simulink model "dual_thyristor_bridge_rectifier"  (R2025b)
settings: Solver=ode1be  StartTime=0.0  StopTime=simlength  FixedStep=tc  MaxStep=tc
values from neighbouring files (symbols this model uses):
  n1 = 35    [voltage_spectrum_analysis.m]
  omega_grid_emulator_nom = w_grid    (= 314.159265359)    [grid_emulator.m]
  vn_eta_pu = 0    [grid_emulator.m]
  vn_xi_pu = 0    [grid_emulator.m]
  vp_xi_pu = 1    [grid_emulator.m]
  w_grid = f_grid*2*pi    (= 314.159265359)    [grid_emulator.m]
undefined symbols (not defined in the file or in its folder): CSF_11, CSF_13, CSF_5, CSF_7, delta_fht1, Idc_traction_normalization_factor, ki_u_ctrl, kp_u_ctrl, Ld_fht1, LFu_dc, LSF_11, LSF_13, LSF_5, LSF_7, magnitude, n10, omega_fht1, pll_i1, pll_p, RLFu_dc, tc, Tcontrol_rect, ts_ctrl_rect, ugrid_factor, Vdc_traction_normalization_factor, Vgrid_phase_normalization_factor
libraries: fl_lib x299, nesl_utility x67, ee_lib x24, single_phase_transformer_lib x3, cstblocks x3
(part 6 of 6)

== system dual_thyristor_bridge_rectifier/dual_rectifier_bridge/neg_bridge/firing3/oscillator ==
  Data Type Conversion : DataTypeConversion  OutDataTypeStr=double  SaturateOnIntegerOverflow=off  RndMeth=Floor
  Logical Operator1 : Logic  Operator=NOT  AllPortsSameDT=off  OutDataTypeStr=boolean
  Rate Transition : RateTransition  OutPortSampleTime=ts
  Simulink-PS Converter : nesl_utility/Simulink-PS Converter  PhysicalDomain=network_engine_domain  SubClassName=ps_input  LeftPortType=input  RightPortType=output  PseudoPeriodic=off  Frequencies=[]  NoiseDistribution=none  NoiseParameters=[]  Unit=1  AffineConversion=off  FilteringAndDerivatives=provide  SimscapeFilterOrder=1  InputFilterTimeConstant=0.001  UdotUserProvided=0
  Unit Delay1 : UnitDelay  SampleTime=Tcontrol_rect  HasFrameUpgradeWarning=on
  output : PMIOPort  Side=Right
  wires:
  Data Type Conversion/1 -> Rate Transition/1
  Unit Delay1/1 -> Logical Operator1/1
  Logical Operator1/1 -> Unit Delay1/1, Data Type Conversion/1
  Rate Transition/1 -> Simulink-PS Converter/1
  connections:
  Simulink-PS Converter/RConn1 -- output/RConn1

== system dual_thyristor_bridge_rectifier/dual_rectifier_bridge/neg_bridge/firing4/oscillator ==
  Data Type Conversion : DataTypeConversion  OutDataTypeStr=double  SaturateOnIntegerOverflow=off  RndMeth=Floor
  Logical Operator1 : Logic  Operator=NOT  AllPortsSameDT=off  OutDataTypeStr=boolean
  Rate Transition : RateTransition  OutPortSampleTime=ts
  Simulink-PS Converter : nesl_utility/Simulink-PS Converter  PhysicalDomain=network_engine_domain  SubClassName=ps_input  LeftPortType=input  RightPortType=output  PseudoPeriodic=off  Frequencies=[]  NoiseDistribution=none  NoiseParameters=[]  Unit=1  AffineConversion=off  FilteringAndDerivatives=provide  SimscapeFilterOrder=1  InputFilterTimeConstant=0.001  UdotUserProvided=0
  Unit Delay1 : UnitDelay  SampleTime=Tcontrol_rect  HasFrameUpgradeWarning=on
  output : PMIOPort  Side=Right
  wires:
  Logical Operator1/1 -> Unit Delay1/1, Data Type Conversion/1
  Unit Delay1/1 -> Logical Operator1/1
  Data Type Conversion/1 -> Rate Transition/1
  Rate Transition/1 -> Simulink-PS Converter/1
  connections:
  Simulink-PS Converter/RConn1 -- output/RConn1

== system dual_thyristor_bridge_rectifier/dual_rectifier_bridge/neg_bridge/firing5/oscillator ==
  Data Type Conversion : DataTypeConversion  OutDataTypeStr=double  SaturateOnIntegerOverflow=off  RndMeth=Floor
  Logical Operator1 : Logic  Operator=NOT  AllPortsSameDT=off  OutDataTypeStr=boolean
  Rate Transition : RateTransition  OutPortSampleTime=ts
  Simulink-PS Converter : nesl_utility/Simulink-PS Converter  PhysicalDomain=network_engine_domain  SubClassName=ps_input  LeftPortType=input  RightPortType=output  PseudoPeriodic=off  Frequencies=[]  NoiseDistribution=none  NoiseParameters=[]  Unit=1  AffineConversion=off  FilteringAndDerivatives=provide  SimscapeFilterOrder=1  InputFilterTimeConstant=0.001  UdotUserProvided=0
  Unit Delay1 : UnitDelay  SampleTime=Tcontrol_rect  HasFrameUpgradeWarning=on
  output : PMIOPort  Side=Right
  wires:
  Data Type Conversion/1 -> Rate Transition/1
  Unit Delay1/1 -> Logical Operator1/1
  Logical Operator1/1 -> Unit Delay1/1, Data Type Conversion/1
  Rate Transition/1 -> Simulink-PS Converter/1
  connections:
  Simulink-PS Converter/RConn1 -- output/RConn1

== system dual_thyristor_bridge_rectifier/dual_rectifier_bridge/neg_bridge/firing6/oscillator ==
  Data Type Conversion : DataTypeConversion  OutDataTypeStr=double  SaturateOnIntegerOverflow=off  RndMeth=Floor
  Logical Operator1 : Logic  Operator=NOT  AllPortsSameDT=off  OutDataTypeStr=boolean
  Rate Transition : RateTransition  OutPortSampleTime=ts
  Simulink-PS Converter : nesl_utility/Simulink-PS Converter  PhysicalDomain=network_engine_domain  SubClassName=ps_input  LeftPortType=input  RightPortType=output  PseudoPeriodic=off  Frequencies=[]  NoiseDistribution=none  NoiseParameters=[]  Unit=1  AffineConversion=off  FilteringAndDerivatives=provide  SimscapeFilterOrder=1  InputFilterTimeConstant=0.001  UdotUserProvided=0
  Unit Delay1 : UnitDelay  SampleTime=Tcontrol_rect  HasFrameUpgradeWarning=on
  output : PMIOPort  Side=Right
  wires:
  Logical Operator1/1 -> Data Type Conversion/1, Unit Delay1/1
  Unit Delay1/1 -> Logical Operator1/1
  Data Type Conversion/1 -> Rate Transition/1
  Rate Transition/1 -> Simulink-PS Converter/1
  connections:
  Simulink-PS Converter/RConn1 -- output/RConn1

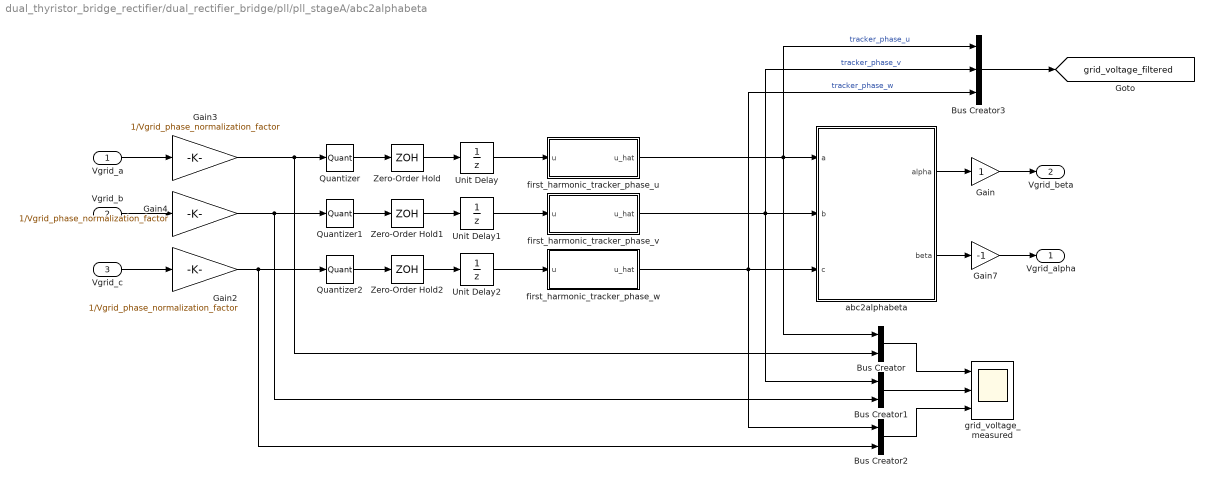
== system dual_thyristor_bridge_rectifier/dual_rectifier_bridge/pll/pll_stageA/abc2alphabeta ==
  Vgrid_a : Inport
  Vgrid_b : Inport  Port=2
  Vgrid_c : Inport  Port=3
  Bus Creator : BusCreator  Inputs=2
  Bus Creator1 : BusCreator  Inputs=2
  Bus Creator2 : BusCreator  Inputs=2
  Bus Creator3 : BusCreator  Inputs=3
  Gain : Gain
  Gain2 : Gain  Gain=1/Vgrid_phase_normalization_factor
  Gain3 : Gain  Gain=1/Vgrid_phase_normalization_factor
  Gain4 : Gain  Gain=1/Vgrid_phase_normalization_factor
  Gain7 : Gain  Gain=-1
  Quantizer : Quantizer  QuantizationInterval=2^-11
  Quantizer1 : Quantizer  QuantizationInterval=2^-11
  Quantizer2 : Quantizer  QuantizationInterval=2^-11
  Unit Delay : UnitDelay  SampleTime=ts_ctrl_rect  HasFrameUpgradeWarning=on
  Unit Delay1 : UnitDelay  SampleTime=ts_ctrl_rect  HasFrameUpgradeWarning=on
  Unit Delay2 : UnitDelay  SampleTime=ts_ctrl_rect  HasFrameUpgradeWarning=on
  Zero-Order Hold : ZeroOrderHold  SampleTime=ts_ctrl_rect
  Zero-Order Hold1 : ZeroOrderHold  SampleTime=ts_ctrl_rect
  Zero-Order Hold2 : ZeroOrderHold  SampleTime=ts_ctrl_rect
  abc2alphabeta : Subsystem
  first_harmonic_tracker_phase_u : Subsystem
  first_harmonic_tracker_phase_v : Subsystem
  first_harmonic_tracker_phase_w : Subsystem
  grid_voltage_measured : Scope  NumInputPorts=3
      settings: SampleTime=ts_ctrl_rect  ActiveDisplayYMinimum=-1.64432  ActiveDisplayYMaximum=1.33618
  Vgrid_alpha : Outport
  Vgrid_beta : Outport  Port=2
  tag scope: grid_voltage_filtered=global
  wires:
  Vgrid_a/1 -> Gain3/1
  Vgrid_b/1 -> Gain4/1
  Vgrid_c/1 -> Gain2/1
  abc2alphabeta/2("beta ") -> Gain7/1
  abc2alphabeta/1("alpha ") -> Gain/1
  Gain/1 -> Vgrid_beta/1
  Gain7/1 -> Vgrid_alpha/1
  Zero-Order Hold/1 -> Unit Delay/1
  Zero-Order Hold1/1 -> Unit Delay1/1
  Zero-Order Hold2/1 -> Unit Delay2/1
  Bus Creator3/1 -> [grid_voltage_filtered]
  Bus Creator/1 -> grid_voltage_measured/1
  Bus Creator1/1 -> grid_voltage_measured/2
  Bus Creator2/1 -> grid_voltage_measured/3
  first_harmonic_tracker_phase_u/1(u_hat) -> Bus Creator/1, Bus Creator3/1, abc2alphabeta/1(a)  "tracker_phase_u"
  first_harmonic_tracker_phase_v/1(u_hat) -> Bus Creator1/1, Bus Creator3/2, abc2alphabeta/2(b)  "tracker_phase_v"
  first_harmonic_tracker_phase_w/1(u_hat) -> Bus Creator2/1, abc2alphabeta/3(c), Bus Creator3/3  "tracker_phase_w"
  Unit Delay1/1 -> first_harmonic_tracker_phase_v/1(u)
  Unit Delay/1 -> first_harmonic_tracker_phase_u/1(u)
  Unit Delay2/1 -> first_harmonic_tracker_phase_w/1(u)
  Gain3/1 -> Quantizer/1, Bus Creator/2
  Gain4/1 -> Quantizer1/1, Bus Creator1/2
  Gain2/1 -> Quantizer2/1, Bus Creator2/2
  Quantizer2/1 -> Zero-Order Hold2/1
  Quantizer1/1 -> Zero-Order Hold1/1
  Quantizer/1 -> Zero-Order Hold/1

== system dual_thyristor_bridge_rectifier/dual_rectifier_bridge/pll/pll_stageB/alphabeta2xieta ==
  alpha : Inport
  beta : Inport  Port=2
  wt : Inport  Port=3
  Product{,1..3} (4 alike) : Product  RndMeth=Zero
  Sum : Sum
  Sum1 : Sum  Inputs=-+
  Trigonometric Function : Trigonometry  Operator=cos
  Trigonometric Function1 : Trigonometry
  xi : Outport
  eta : Outport  Port=2
  wires:
  Trigonometric Function/1 -> [cos]
  Trigonometric Function1/1 -> [sin]
  wt/1 -> Trigonometric Function1/1, Trigonometric Function/1
  Sum1/1 -> eta/1
  Sum/1 -> xi/1
  [cos] -> Product3/1
  Product3/1 -> Sum1/2
  Product2/1 -> Sum1/1
  [sin] -> Product2/1
  beta/1 -> Product3/2, Product1/2
  [sin] -> Product1/1
  Product1/1 -> Sum/2
  Product/1 -> Sum/1
  alpha/1 -> Product2/2, Product/2
  [cos] -> Product/1

== system dual_thyristor_bridge_rectifier/dual_rectifier_bridge/pll/pll_stageB/pll_2 ==
  eta : Inport
  -2<x<2 : Saturate  UpperLimit=2  LowerLimit=-2
  Constant1 : Constant  Value=2*pi
  Constant3 : Constant  Value=0
  Constant4 : Constant  Value=w_grid
  Constant7 : Constant
  Math Function1 : Math  Operator=mod  SignedPower=on
  Product1 : Product  RndMeth=Zero
  Product2 : Product  RndMeth=Zero
  Sum1 : Sum  Inputs=|-+
  Sum3 : Sum  SaturateOnIntegerOverflow=on
  Sum4 : Sum  SaturateOnIntegerOverflow=on
  Sum5 : Sum  Inputs=+++
  Unit Delay1 : UnitDelay  SampleTime=ts_ctrl_rect  HasFrameUpgradeWarning=on
  Unit Delay4 : UnitDelay  SampleTime=ts_ctrl_rect  HasFrameUpgradeWarning=on
  kp : Gain  Gain=pll_i1*ts_ctrl_rect  SaturateOnIntegerOverflow=on  OutDataTypeStr=Inherit: Same as input  ParamDataTypeStr=Inherit: Same as input
  kp1 : Gain  Gain=pll_p  SaturateOnIntegerOverflow=on  OutDataTypeStr=Inherit: Same as input  ParamDataTypeStr=Inherit: Same as input
  kp2 : Gain  Gain=ts_ctrl_rect  SaturateOnIntegerOverflow=on  OutDataTypeStr=Inherit: Same as input  ParamDataTypeStr=Inherit: Same as input
  kp3 : Gain  Gain=-1  SaturateOnIntegerOverflow=on  OutDataTypeStr=Inherit: Same as input  ParamDataTypeStr=Inherit: Same as input
  theta_est : Outport
  wires:
  Constant7/1 -> Sum5/3
  Constant3/1 -> Sum1/2
  [Vgrid_unorm_posneg] -> Product1/2
  Product2/1 -> kp2/1
  kp/1 -> Sum3/1
  Sum4/1 -> Math Function1/1
  kp1/1 -> Sum5/1
  Product1/1 -> Sum1/1
  Sum1/1 -> kp3/1
  Math Function1/1 -> theta_est/1, Unit Delay1/1
  -2<x<2/1 -> Unit Delay4/1, Sum5/2  "i1"
  Unit Delay4/1 -> Sum3/2
  Sum3/1 -> -2<x<2/1
  kp2/1 -> Sum4/1
  Sum5/1 -> Product2/1
  Constant4/1 -> Product2/2
  Unit Delay1/1 -> Sum4/2
  Constant1/1 -> Math Function1/2
  eta/1 -> Product1/1
  kp3/1 -> kp/1, kp1/1

== system dual_thyristor_bridge_rectifier/dual_rectifier_bridge/pos_bridge/firing1/oscillator ==
  Data Type Conversion : DataTypeConversion  OutDataTypeStr=double  SaturateOnIntegerOverflow=off  RndMeth=Floor
  Logical Operator1 : Logic  Operator=NOT  AllPortsSameDT=off  OutDataTypeStr=boolean
  Rate Transition : RateTransition  OutPortSampleTime=ts
  Simulink-PS Converter : nesl_utility/Simulink-PS Converter  PhysicalDomain=network_engine_domain  SubClassName=ps_input  LeftPortType=input  RightPortType=output  PseudoPeriodic=off  Frequencies=[]  NoiseDistribution=none  NoiseParameters=[]  Unit=1  AffineConversion=off  FilteringAndDerivatives=provide  SimscapeFilterOrder=1  InputFilterTimeConstant=0.001  UdotUserProvided=0
  Unit Delay1 : UnitDelay  SampleTime=Tcontrol_rect  HasFrameUpgradeWarning=on
  output : PMIOPort  Side=Right
  wires:
  Rate Transition/1 -> Simulink-PS Converter/1
  Logical Operator1/1 -> Data Type Conversion/1, Unit Delay1/1
  Unit Delay1/1 -> Logical Operator1/1
  Data Type Conversion/1 -> Rate Transition/1
  connections:
  Simulink-PS Converter/RConn1 -- output/RConn1

== system dual_thyristor_bridge_rectifier/dual_rectifier_bridge/pos_bridge/firing2/oscillator ==
  Data Type Conversion : DataTypeConversion  OutDataTypeStr=double  SaturateOnIntegerOverflow=off  RndMeth=Floor
  Logical Operator1 : Logic  Operator=NOT  AllPortsSameDT=off  OutDataTypeStr=boolean
  Rate Transition : RateTransition  OutPortSampleTime=ts
  Simulink-PS Converter : nesl_utility/Simulink-PS Converter  PhysicalDomain=network_engine_domain  SubClassName=ps_input  LeftPortType=input  RightPortType=output  PseudoPeriodic=off  Frequencies=[]  NoiseDistribution=none  NoiseParameters=[]  Unit=1  AffineConversion=off  FilteringAndDerivatives=provide  SimscapeFilterOrder=1  InputFilterTimeConstant=0.001  UdotUserProvided=0
  Unit Delay1 : UnitDelay  SampleTime=Tcontrol_rect  HasFrameUpgradeWarning=on
  output : PMIOPort  Side=Right
  wires:
  Rate Transition/1 -> Simulink-PS Converter/1
  Data Type Conversion/1 -> Rate Transition/1
  Unit Delay1/1 -> Logical Operator1/1
  Logical Operator1/1 -> Unit Delay1/1, Data Type Conversion/1
  connections:
  Simulink-PS Converter/RConn1 -- output/RConn1

== system dual_thyristor_bridge_rectifier/dual_rectifier_bridge/pos_bridge/firing3/oscillator ==
  Data Type Conversion : DataTypeConversion  OutDataTypeStr=double  SaturateOnIntegerOverflow=off  RndMeth=Floor
  Logical Operator1 : Logic  Operator=NOT  AllPortsSameDT=off  OutDataTypeStr=boolean
  Rate Transition : RateTransition  OutPortSampleTime=ts
  Simulink-PS Converter : nesl_utility/Simulink-PS Converter  PhysicalDomain=network_engine_domain  SubClassName=ps_input  LeftPortType=input  RightPortType=output  PseudoPeriodic=off  Frequencies=[]  NoiseDistribution=none  NoiseParameters=[]  Unit=1  AffineConversion=off  FilteringAndDerivatives=provide  SimscapeFilterOrder=1  InputFilterTimeConstant=0.001  UdotUserProvided=0
  Unit Delay1 : UnitDelay  SampleTime=Tcontrol_rect  HasFrameUpgradeWarning=on
  output : PMIOPort  Side=Right
  wires:
  Rate Transition/1 -> Simulink-PS Converter/1
  Logical Operator1/1 -> Data Type Conversion/1, Unit Delay1/1
  Unit Delay1/1 -> Logical Operator1/1
  Data Type Conversion/1 -> Rate Transition/1
  connections:
  Simulink-PS Converter/RConn1 -- output/RConn1

== system dual_thyristor_bridge_rectifier/dual_rectifier_bridge/pos_bridge/firing4/oscillator ==
  Data Type Conversion : DataTypeConversion  OutDataTypeStr=double  SaturateOnIntegerOverflow=off  RndMeth=Floor
  Logical Operator1 : Logic  Operator=NOT  AllPortsSameDT=off  OutDataTypeStr=boolean
  Rate Transition : RateTransition  OutPortSampleTime=ts
  Simulink-PS Converter : nesl_utility/Simulink-PS Converter  PhysicalDomain=network_engine_domain  SubClassName=ps_input  LeftPortType=input  RightPortType=output  PseudoPeriodic=off  Frequencies=[]  NoiseDistribution=none  NoiseParameters=[]  Unit=1  AffineConversion=off  FilteringAndDerivatives=provide  SimscapeFilterOrder=1  InputFilterTimeConstant=0.001  UdotUserProvided=0
  Unit Delay1 : UnitDelay  SampleTime=Tcontrol_rect  HasFrameUpgradeWarning=on
  output : PMIOPort  Side=Right
  wires:
  Rate Transition/1 -> Simulink-PS Converter/1
  Data Type Conversion/1 -> Rate Transition/1
  Unit Delay1/1 -> Logical Operator1/1
  Logical Operator1/1 -> Data Type Conversion/1, Unit Delay1/1
  connections:
  Simulink-PS Converter/RConn1 -- output/RConn1

== system dual_thyristor_bridge_rectifier/dual_rectifier_bridge/pos_bridge/firing5/oscillator ==
  Data Type Conversion : DataTypeConversion  OutDataTypeStr=double  SaturateOnIntegerOverflow=off  RndMeth=Floor
  Logical Operator1 : Logic  Operator=NOT  AllPortsSameDT=off  OutDataTypeStr=boolean
  Rate Transition : RateTransition  OutPortSampleTime=ts
  Simulink-PS Converter : nesl_utility/Simulink-PS Converter  PhysicalDomain=network_engine_domain  SubClassName=ps_input  LeftPortType=input  RightPortType=output  PseudoPeriodic=off  Frequencies=[]  NoiseDistribution=none  NoiseParameters=[]  Unit=1  AffineConversion=off  FilteringAndDerivatives=provide  SimscapeFilterOrder=1  InputFilterTimeConstant=0.001  UdotUserProvided=0
  Unit Delay1 : UnitDelay  SampleTime=Tcontrol_rect  HasFrameUpgradeWarning=on
  output : PMIOPort  Side=Right
  wires:
  Rate Transition/1 -> Simulink-PS Converter/1
  Logical Operator1/1 -> Data Type Conversion/1, Unit Delay1/1
  Unit Delay1/1 -> Logical Operator1/1
  Data Type Conversion/1 -> Rate Transition/1
  connections:
  Simulink-PS Converter/RConn1 -- output/RConn1

== system dual_thyristor_bridge_rectifier/dual_rectifier_bridge/pos_bridge/firing6/oscillator ==
  Data Type Conversion : DataTypeConversion  OutDataTypeStr=double  SaturateOnIntegerOverflow=off  RndMeth=Floor
  Logical Operator1 : Logic  Operator=NOT  AllPortsSameDT=off  OutDataTypeStr=boolean
  Rate Transition : RateTransition  OutPortSampleTime=ts
  Simulink-PS Converter : nesl_utility/Simulink-PS Converter  PhysicalDomain=network_engine_domain  SubClassName=ps_input  LeftPortType=input  RightPortType=output  PseudoPeriodic=off  Frequencies=[]  NoiseDistribution=none  NoiseParameters=[]  Unit=1  AffineConversion=off  FilteringAndDerivatives=provide  SimscapeFilterOrder=1  InputFilterTimeConstant=0.001  UdotUserProvided=0
  Unit Delay1 : UnitDelay  SampleTime=Tcontrol_rect  HasFrameUpgradeWarning=on
  output : PMIOPort  Side=Right
  wires:
  Rate Transition/1 -> Simulink-PS Converter/1
  Data Type Conversion/1 -> Rate Transition/1
  Unit Delay1/1 -> Logical Operator1/1
  Logical Operator1/1 -> Unit Delay1/1, Data Type Conversion/1
  connections:
  Simulink-PS Converter/RConn1 -- output/RConn1

== system dual_thyristor_bridge_rectifier/grid/grid_emulator/grid_emulator/phase_gen ==
  Constant4 : Constant  Value=omega_grid_emulator_nom
  Integrator : Integrator
  bounder1 : MATLAB Function  TreatAsAtomicUnit=on  SystemSampleTime=ts_ctrl_rect
  grid_emu_phase : Outport  VectorParamsAs1DForOutWhenUnconnected=off
  tag scope: gamma_grid_emulator=global
  wires:
  bounder1/1(y) -> [gamma_grid_emulator], grid_emu_phase/1  "grid_emu_phase"
  Constant4/1 -> Integrator/1
  Integrator/1 -> bounder1/1(u)

== system dual_thyristor_bridge_rectifier/grid/grid_emulator/grid_emulator/voltage_reference ==
  grid_emu_phase : Inport
  Vxi_p : Inport  Port=2
  Vxi_n : Inport  Port=3
  Veta_n : Inport  Port=4
  Constant2 : Constant  Value=0
  Sum1 : Sum  Inputs=|++
  Sum4 : Sum  Inputs=|++
  alphabeta2abc : MATLAB Function  TreatAsAtomicUnit=on  SystemSampleTime=ts_ctrl_rect
  xieta2alphabeta_neg : MATLAB Function  TreatAsAtomicUnit=on  SystemSampleTime=ts_ctrl_rect
  xieta2alphabeta_pos : MATLAB Function  TreatAsAtomicUnit=on  SystemSampleTime=ts_ctrl_rect
  V1_ref : Outport  VectorParamsAs1DForOutWhenUnconnected=off
  V2_ref : Outport  Port=2  VectorParamsAs1DForOutWhenUnconnected=off
  V3_ref : Outport  Port=3  VectorParamsAs1DForOutWhenUnconnected=off
  wires:
  xieta2alphabeta_pos/1(alpha) -> Sum1/1
  Sum1/1 -> alphabeta2abc/1(alpha)
  xieta2alphabeta_pos/2(beta) -> Sum4/1
  Sum4/1 -> alphabeta2abc/2(beta)
  xieta2alphabeta_neg/1(alpha) -> Sum1/2
  xieta2alphabeta_neg/2(beta) -> Sum4/2
  grid_emu_phase/1 -> xieta2alphabeta_neg/3(gamma), xieta2alphabeta_pos/3(gamma)
  Vxi_p/1 -> xieta2alphabeta_pos/1(xi)
  Constant2/1 -> xieta2alphabeta_pos/2(eta)
  Vxi_n/1 -> xieta2alphabeta_neg/1(xi)
  Veta_n/1 -> xieta2alphabeta_neg/2(eta)
  alphabeta2abc/1(a) -> V1_ref/1
  alphabeta2abc/2(b) -> V2_ref/1
  alphabeta2abc/3(c) -> V3_ref/1

== system dual_thyristor_bridge_rectifier/grid/grid_emulator/grid_emulator/voltage_source ==
  Constant : Constant  Value=vp_xi_pu
  Constant1 : Constant  Value=vn_xi_pu
  Constant2 : Constant  Value=vn_eta_pu
  Gain1 : Gain  Gain=Vgrid_phase_normalization_factor
  Gain2 : Gain  Gain=ugrid_factor
  Gain3 : Gain  Gain=ugrid_factor
  Gain4 : Gain  Gain=ugrid_factor
  Gain7 : Gain  Gain=Vgrid_phase_normalization_factor
  Gain8 : Gain  Gain=Vgrid_phase_normalization_factor
  LTI System1 : cstblocks/LTI System  sys=LPF1_ss_c  IC=[0]  PadeOrder=0
  LTI System2 : cstblocks/LTI System  sys=LPF1_ss_c  IC=[0]  PadeOrder=0
  LTI System6 : cstblocks/LTI System  sys=LPF1_ss_c  IC=[0]  PadeOrder=0
  vp_xi : Outport  VectorParamsAs1DForOutWhenUnconnected=off
  vn_xi : Outport  Port=2  VectorParamsAs1DForOutWhenUnconnected=off
  vn_eta : Outport  Port=3  VectorParamsAs1DForOutWhenUnconnected=off
  wires:
  LTI System2/1 -> Gain7/1
  LTI System1/1 -> Gain8/1
  Gain7/1 -> Gain2/1
  Gain8/1 -> Gain3/1
  Gain1/1 -> Gain4/1
  LTI System6/1 -> Gain1/1
  Gain2/1 -> vp_xi/1
  Gain3/1 -> vn_xi/1
  Gain4/1 -> vn_eta/1
  Constant/1 -> LTI System2/1
  Constant1/1 -> LTI System1/1
  Constant2/1 -> LTI System6/1

== system dual_thyristor_bridge_rectifier/dual_rectifier_bridge/pll/pll_stageA/abc2alphabeta/abc2alphabeta ==
  a : Inport
  b : Inport  Port=2
  c : Inport  Port=3
  Gain1 : Gain  Gain=-1/2
  Gain11 : Gain  Gain=-1/2
  Gain2 : Gain  Gain=0
  Gain3 : Gain  Gain=-sqrt(3)/2
  Gain4 : Gain  Gain=sqrt(3)/2
  Gain8 : Gain  Gain=2/3
  Gain9 : Gain  Gain=2/3
  Sum : Sum  Inputs=+++
  Sum1 : Sum  Inputs=+++
  "alpha " : Outport
  "beta " : Outport  Port=2
  wires:
  Sum1/1 -> Gain9/1
  Sum/1 -> Gain8/1
  Gain4/1 -> Sum/2
  Gain2/1 -> Sum/1
  a/1 -> Gain2/1, Sum1/1
  Gain3/1 -> Sum/3
  b/1 -> Gain4/1, Gain11/1
  c/1 -> Gain3/1, Gain1/1
  Gain1/1 -> Sum1/3
  Gain11/1 -> Sum1/2
  Gain9/1 -> "alpha "/1
  Gain8/1 -> "beta "/1

== system dual_thyristor_bridge_rectifier/dual_rectifier_bridge/pll/pll_stageA/abc2alphabeta/first_harmonic_tracker_phase_u ==
  u : Inport
  Bus Selector : BusSelector  OutputSignals=output_pu_hat
  C Caller : CCaller  FunctionName=first_harmonic_tracker_process_simulink  PortSpecificationStruct="%)30     .    B \\   8    (     @         %    \"     D    !     0         %  0 \"0    $    _    07)G3F%M90  4&]R=$YA;64 4V-O<&4     26YD97@     5'EP90      4VEZ90      27-';&]B86P   X    P    !@    @    $          4    (     0    ,    !         !   P!O=70 #@   #     &    \"     0         !0    @    !     P    $         $  # &]U=  .    .     8    (    !          %    \"     $    &     0         0  ...(+4988 chars)"  SampleTime=ts_ctrl_rect
  Constant : Constant  Value=ts_ctrl_rect
  Constant1 : Constant  Value=0
  Constant4 : Constant  Value=omega_fht1
  Constant5 : Constant  Value=delta_fht1
  Constant6 : Constant  Value=Ld_fht1(1)
  Constant7 : Constant  Value=Ld_fht1(2)
  Data Type Conversion{1..2,6..9} (6 alike) : DataTypeConversion  OutDataTypeStr=single  SaturateOnIntegerOverflow=off  RndMeth=Floor
  Data Type Conversion3 : DataTypeConversion  OutDataTypeStr=uint8  SaturateOnIntegerOverflow=off  RndMeth=Floor
  Data Type Conversion4 : DataTypeConversion  OutDataTypeStr=double  SaturateOnIntegerOverflow=off  RndMeth=Floor
  Data Type Conversion5 : DataTypeConversion  OutDataTypeStr=uint8  SaturateOnIntegerOverflow=off  RndMeth=Floor
  Step : Step  Time=ts_ctrl_rect  Before=1  After=0  SampleTime=ts_ctrl_rect
  Zero-Order Hold{,1..7} (8 alike) : ZeroOrderHold  SampleTime=ts_ctrl_rect
  u_hat : Outport
  wires:
  Data Type Conversion4/1 -> u_hat/1
  Data Type Conversion3/1 -> C Caller/1
  Data Type Conversion2/1 -> C Caller/2
  C Caller/1 -> Bus Selector/1
  Bus Selector/1 -> Data Type Conversion4/1  "<output_pu_hat>"
  Step/1 -> Zero-Order Hold/1
  u/1 -> Zero-Order Hold1/1
  Constant/1 -> Zero-Order Hold2/1
  Constant1/1 -> Zero-Order Hold3/1
  Zero-Order Hold/1 -> Data Type Conversion3/1
  Zero-Order Hold1/1 -> Data Type Conversion2/1
  Zero-Order Hold2/1 -> Data Type Conversion1/1
  Zero-Order Hold3/1 -> Data Type Conversion5/1
  Constant4/1 -> Zero-Order Hold4/1
  Constant6/1 -> Zero-Order Hold6/1
  Constant7/1 -> Zero-Order Hold7/1
  Constant5/1 -> Zero-Order Hold5/1
  Data Type Conversion1/1 -> C Caller/3
  Data Type Conversion5/1 -> C Caller/8
  Data Type Conversion6/1 -> C Caller/4
  Data Type Conversion7/1 -> C Caller/5
  Data Type Conversion8/1 -> C Caller/6
  Data Type Conversion9/1 -> C Caller/7
  Zero-Order Hold4/1 -> Data Type Conversion6/1
  Zero-Order Hold5/1 -> Data Type Conversion7/1
  Zero-Order Hold6/1 -> Data Type Conversion8/1
  Zero-Order Hold7/1 -> Data Type Conversion9/1

== system dual_thyristor_bridge_rectifier/dual_rectifier_bridge/pll/pll_stageA/abc2alphabeta/first_harmonic_tracker_phase_v ==
  u : Inport
  Bus Selector : BusSelector  OutputSignals=output_pu_hat
  C Caller : CCaller  FunctionName=first_harmonic_tracker_process_simulink  PortSpecificationStruct="%)30     .    V @   8    (     @         %    \"     4    !     0         %  0 \"0    $    _    07)G3F%M90  4&]R=$YA;64 4V-O<&4     26YD97@     5'EP90      4VEZ90      27-';&]B86P   X    P    !@    @    $          4    (     0    ,    !         !   P!O=70 #@   #     &    \"     0         !0    @    !     P    $         $  # &]U=  .    .     8    (    !          %    \"     $    &     0         0   ...(+2669 chars)"  SampleTime=ts_ctrl_rect
  Constant : Constant  Value=ts_ctrl_rect
  Constant1 : Constant  Value=2
  Data Type Conversion1 : DataTypeConversion  OutDataTypeStr=single  SaturateOnIntegerOverflow=off  RndMeth=Floor
  Data Type Conversion2 : DataTypeConversion  OutDataTypeStr=single  SaturateOnIntegerOverflow=off  RndMeth=Floor
  Data Type Conversion3 : DataTypeConversion  OutDataTypeStr=uint8  SaturateOnIntegerOverflow=off  RndMeth=Floor
  Data Type Conversion4 : DataTypeConversion  OutDataTypeStr=double  SaturateOnIntegerOverflow=off  RndMeth=Floor
  Data Type Conversion5 : DataTypeConversion  OutDataTypeStr=uint8  SaturateOnIntegerOverflow=off  RndMeth=Floor
  Step : Step  Time=ts_ctrl_rect  Before=1  After=0  SampleTime=ts_ctrl_rect
  Zero-Order Hold{,1..3} (4 alike) : ZeroOrderHold  SampleTime=ts_ctrl_rect
  u_hat : Outport
  wires:
  Constant1/1 -> Zero-Order Hold3/1
  Data Type Conversion5/1 -> C Caller/4
  Constant/1 -> Zero-Order Hold2/1
  u/1 -> Zero-Order Hold1/1
  Step/1 -> Zero-Order Hold/1
  Bus Selector/1 -> Data Type Conversion4/1  "<output_pu_hat>"
  C Caller/1 -> Bus Selector/1
  Data Type Conversion2/1 -> C Caller/2
  Data Type Conversion1/1 -> C Caller/3
  Data Type Conversion3/1 -> C Caller/1
  Data Type Conversion4/1 -> u_hat/1
  Zero-Order Hold/1 -> Data Type Conversion3/1
  Zero-Order Hold1/1 -> Data Type Conversion2/1
  Zero-Order Hold2/1 -> Data Type Conversion1/1
  Zero-Order Hold3/1 -> Data Type Conversion5/1

== system dual_thyristor_bridge_rectifier/dual_rectifier_bridge/pll/pll_stageA/abc2alphabeta/first_harmonic_tracker_phase_w ==
  u : Inport
  Bus Selector : BusSelector  OutputSignals=output_pu_hat
  C Caller : CCaller  FunctionName=first_harmonic_tracker_process_simulink  PortSpecificationStruct="%)30     .    V @   8    (     @         %    \"     4    !     0         %  0 \"0    $    _    07)G3F%M90  4&]R=$YA;64 4V-O<&4     26YD97@     5'EP90      4VEZ90      27-';&]B86P   X    P    !@    @    $          4    (     0    ,    !         !   P!O=70 #@   #     &    \"     0         !0    @    !     P    $         $  # &]U=  .    .     8    (    !          %    \"     $    &     0         0   ...(+2669 chars)"  SampleTime=ts_ctrl_rect
  Constant : Constant  Value=ts_ctrl_rect
  Constant1 : Constant  Value=4
  Data Type Conversion1 : DataTypeConversion  OutDataTypeStr=single  SaturateOnIntegerOverflow=off  RndMeth=Floor
  Data Type Conversion2 : DataTypeConversion  OutDataTypeStr=single  SaturateOnIntegerOverflow=off  RndMeth=Floor
  Data Type Conversion3 : DataTypeConversion  OutDataTypeStr=uint8  SaturateOnIntegerOverflow=off  RndMeth=Floor
  Data Type Conversion4 : DataTypeConversion  OutDataTypeStr=double  SaturateOnIntegerOverflow=off  RndMeth=Floor
  Data Type Conversion5 : DataTypeConversion  OutDataTypeStr=uint8  SaturateOnIntegerOverflow=off  RndMeth=Floor
  Step : Step  Time=ts_ctrl_rect  Before=1  After=0  SampleTime=ts_ctrl_rect
  Zero-Order Hold{,1..3} (4 alike) : ZeroOrderHold  SampleTime=ts_ctrl_rect
  u_hat : Outport
  wires:
  Data Type Conversion4/1 -> u_hat/1
  Data Type Conversion3/1 -> C Caller/1
  Data Type Conversion1/1 -> C Caller/3
  Data Type Conversion2/1 -> C Caller/2
  C Caller/1 -> Bus Selector/1
  Bus Selector/1 -> Data Type Conversion4/1  "<output_pu_hat>"
  Step/1 -> Zero-Order Hold/1
  u/1 -> Zero-Order Hold1/1
  Constant/1 -> Zero-Order Hold2/1
  Data Type Conversion5/1 -> C Caller/4
  Constant1/1 -> Zero-Order Hold3/1
  Zero-Order Hold/1 -> Data Type Conversion3/1
  Zero-Order Hold1/1 -> Data Type Conversion2/1
  Zero-Order Hold2/1 -> Data Type Conversion1/1
  Zero-Order Hold3/1 -> Data Type Conversion5/1

== matlab function dual_thyristor_bridge_rectifier/grid/grid_emulator/grid_emulator/voltage_reference/alphabeta2abc ==
  data: alpha input; a output; beta input; b output; c output
function [a,b,c] = alphabeta2abc(alpha,beta)

    a  =  alpha;
    b  =  -0.5*alpha + sqrt(3)/2*beta;
    c  =  -0.5*alpha - sqrt(3)/2*beta;
end

== matlab function dual_thyristor_bridge_rectifier/grid/grid_emulator/grid_emulator/voltage_reference/xieta2alphabeta_neg ==
  data: xi input; alpha output; eta input; gamma input; beta output
function [alpha,beta] = xieta2alphabeta_neg(xi,eta,gamma)

    alpha  =  xi*cos(gamma) + eta*sin(gamma);
    beta = -xi*sin(gamma) + eta*cos(gamma);

end

== matlab function dual_thyristor_bridge_rectifier/load_and_control/controller/MATLAB Function1 ==
  data: u input; u_th input; i input; pos output; i_th1 input; i_th2 input; alpha_in input; neg output; alpha_out output; state_out output
function [pos, neg, alpha_out, state_out] = pos_neg_switch(u, u_th, i, i_th1, i_th2, alpha_in)


persistent state
if isempty(state)
    state = 0;
end
    if ((i > i_th1) && (i < i_th2))
        state = 4;
        alpha_out = alpha_in;
        pos = 0;
        neg = 0;
    elseif ((i > i_th1) && (i > i_th2))
        state = 1;
        alpha_out = alpha_in;
        pos = 1;
        neg = 0;
    elseif ((i < -i_th1) && (i > -i_th2))
        state = 2;
        alpha_out = 3.1415 - alpha_in;
        pos = 0;
        neg = 0;
    elseif ((i < -i_th1) && (i < -i_th2))
        state = 3;
        alpha_out = 3.1415 - alpha_in;
        pos = 0;
        neg = 1;
    else
        state = 0;
        alpha_out = alpha_in;
        pos = 0;
        neg = 0;
    end
    state_out = state;
end

== matlab function dual_thyristor_bridge_rectifier/grid/grid_emulator/grid_emulator/voltage_reference/xieta2alphabeta_pos ==
  data: xi input; alpha output; eta input; gamma input; beta output
function [alpha,beta] = xieta2alphabeta_pos(xi,eta,gamma)

    alpha  =  xi*cos(gamma) - eta*sin(gamma);
    beta = xi*sin(gamma) + eta*cos(gamma);

end

== matlab function dual_thyristor_bridge_rectifier/grid/grid_emulator/grid_emulator/phase_gen/bounder1 ==
  data: u input; y output
function y = bounder(u)    
    y = -pi + mod(u+3*pi,2*pi);
end
